simulink model "AirplaneSimModel_SITL_gazebo"  (R2018b)
settings: Solver=ode2  StartTime=0.0  StopTime=inf  FixedStep=0.0025  RelTol=1e-3
undefined symbols (not defined in the file): aileron_left, aileron_right, airplane, alt_ground, atmosphere, elevator, envir, g, htp_trim, rudder, throttle, wind
libraries: unit_conversions_lib x4, ardupilot_sitl_lib x2, conventional_airplane_single_engine_lib x1, atmosphere_lib x1, sensors_lib x1, simulink x1, flightgear_visualization_lib x1
settings Model: Creator=Yannic  LastModifiedBy=yannic
settings OptimizationCC: EfficientMapNaN2IntZero=off
settings HardwareCC: TargetBitPerLong=64  TargetBitPerPointer=64  TargetBitPerSizeT=64  TargetBitPerPtrDiffT=64  TargetLongLongMode=on  TargetIntDivRoundTo=Zero  TargetEndianess=LittleEndian  TargetWordSize=64  TargetHWDeviceType=MATLAB Host  ProdEqTarget=off
settings RTWCC: SystemTargetFile=rsim.tlc  TemplateMakefile=rsim_default_tmf  Description=Rapid Simulation Target  TargetLang=C++  RTWCompilerOptimization=on
settings CodeAppCC: MaxIdLength=128
settings RSimTargetCC: TargetLangStandard=C++03 (ISO)  GeneratePreprocessorConditionals=Use local settings  PreserveStateflowLocalDataDimensions=off

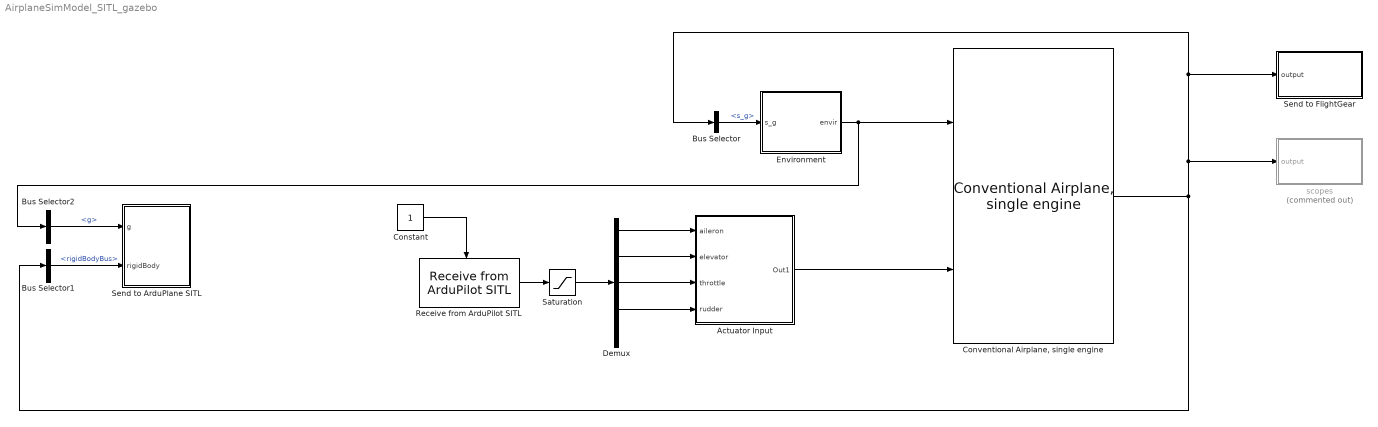
== system AirplaneSimModel_SITL_gazebo ==
  Actuator Input : Subsystem
  Bus Selector : BusSelector  OutputSignals=rigidBodyBus.s_g
  Bus Selector1 : BusSelector  OutputSignals=rigidBodyBus
  Bus Selector2 : BusSelector  OutputSignals=g
  Constant : Constant
  "Conventional Airplane, single engine" : conventional_airplane_single_engine_lib/Conventional Airplane, single engine  airplane=airplane
      settings: SourceProductName=LADAC
  Demux : Demux  Outputs=5
  Environment : Subsystem
  Receive from ArduPilot SITL : ardupilot_sitl_lib/Receive from ArduPilot SITL  idx=[1,2,3,4,5]  IP='127.0.0.1'  Port=9002  sample_time=1/400  blocking_time=1
      settings: SourceProductName=LADAC
  Saturation : Saturate  UpperLimit=1  LowerLimit=0
  Send to ArduPlane SITL : Subsystem
  Send to FlightGear : Subsystem
  scopes : Subsystem  Commented=on
  wires:
  Environment/1(envir) -> Bus Selector2/1, "Conventional Airplane, single engine"/1
  "Conventional Airplane, single engine"/1 -> Bus Selector1/1, Bus Selector/1, Send to FlightGear/1(output), scopes/1(output)
  Bus Selector/1 -> Environment/1(s_g)  "<s_g>"
  Bus Selector1/1 -> Send to ArduPlane SITL/2(rigidBody)  "<rigidBodyBus>"
  Bus Selector2/1 -> Send to ArduPlane SITL/1(g)  "<g>"
  Actuator Input/1(Out1) -> "Conventional Airplane, single engine"/2
  Demux/1 -> Actuator Input/1(aileron)
  Demux/4 -> Actuator Input/4(rudder)
  Receive from ArduPilot SITL/1 -> Saturation/1
  Constant/1 -> Receive from ArduPilot SITL/Enable
  Demux/2 -> Actuator Input/2(elevator)
  Demux/3 -> Actuator Input/3(throttle)
  Saturation/1 -> Demux/1

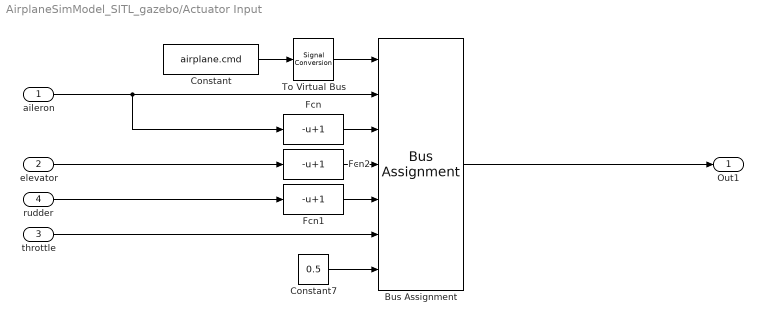
== system AirplaneSimModel_SITL_gazebo/Actuator Input ==
  aileron : Inport
  elevator : Inport  Port=2
  throttle : Inport  Port=3
  rudder : Inport  Port=4
  Bus Assignment : BusAssignment  AssignedSignals=aileron_left,aileron_right,elevator,rudder,throttle,htp_trim
  Constant : Constant  Value=airplane.cmd  OutDataTypeStr=Bus: cmdBus
  Constant7 : Constant  Value=0.5
  Fcn : Fcn  Expr=-u+1
  Fcn1 : Fcn  Expr=-u+1
  Fcn2 : Fcn  Expr=-u+1
  To Virtual Bus : SignalConversion  ConversionOutput=Virtual bus  OverrideOpt=off
  Out1 : Outport
  wires:
  Constant/1 -> To Virtual Bus/1
  Bus Assignment/1 -> Out1/1
  rudder/1 -> Fcn1/1
  elevator/1 -> Fcn2/1
  aileron/1 -> Fcn/1, Bus Assignment/2
  Constant7/1 -> Bus Assignment/7
  Fcn/1 -> Bus Assignment/3
  Fcn1/1 -> Bus Assignment/5
  To Virtual Bus/1 -> Bus Assignment/1
  throttle/1 -> Bus Assignment/6
  Fcn2/1 -> Bus Assignment/4

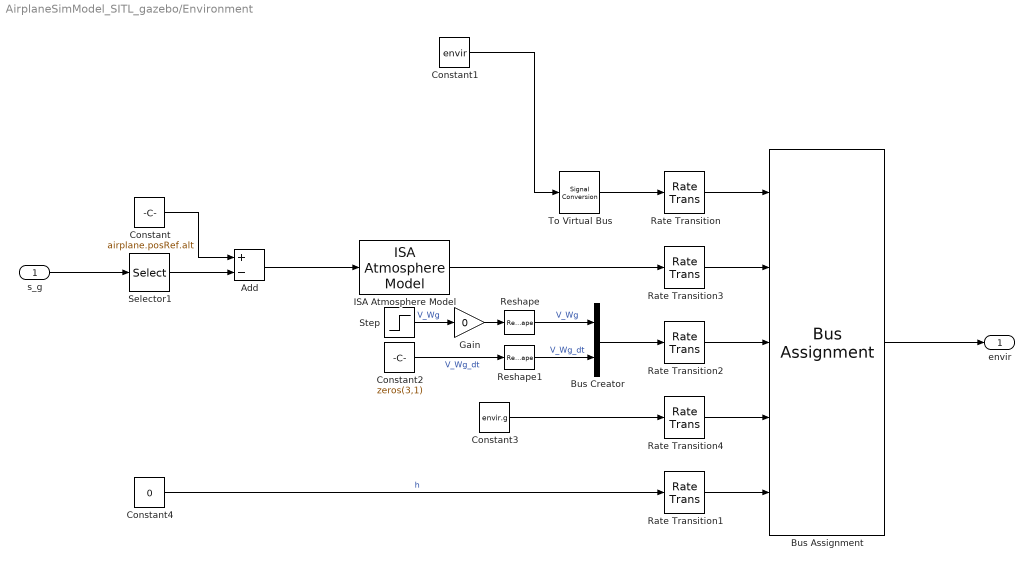
== system AirplaneSimModel_SITL_gazebo/Environment ==
  s_g : Inport
  Add : Sum  Inputs=+-
  Bus Assignment : BusAssignment  AssignedSignals=atmosphere,wind,g,alt_ground
  Bus Creator : BusCreator  Inputs=2
  Constant : Constant  Value=airplane.posRef.alt
  Constant1 : Constant  Value=envir  OutDataTypeStr=Bus: envirBus
  Constant2 : Constant  Value=zeros(3,1)
  Constant3 : Constant  Value=envir.g
  Constant4 : Constant  Value=0
  Gain : Gain  Gain=0
  ISA Atmosphere Model : atmosphere_lib/ISA Atmosphere Model
      settings: SourceProductName=LADAC
  Rate Transition{,1..4} (5 alike) : RateTransition
  Reshape : Reshape  OutputDimensionality=Column vector (2-D)
  Reshape1 : Reshape  OutputDimensionality=Column vector (2-D)
  Selector1 : Selector  InputPortWidth=3  IndexOptions=Index vector (dialog)  Indices=3  OutputSizes=1
  Step : Step  Time=3  After=[0;10;0]  SampleTime=0
  To Virtual Bus : SignalConversion  ConversionOutput=Virtual bus  OverrideOpt=off
  envir : Outport
  wires:
  Constant4/1 -> Rate Transition1/1  "h"
  Rate Transition2/1 -> Bus Assignment/3
  Rate Transition3/1 -> Bus Assignment/2
  Bus Assignment/1 -> envir/1
  Rate Transition/1 -> Bus Assignment/1
  ISA Atmosphere Model/1 -> Rate Transition3/1
  Step/1 -> Gain/1  "V_Wg"
  Rate Transition1/1 -> Bus Assignment/5
  s_g/1 -> Selector1/1
  Bus Creator/1 -> Rate Transition2/1
  Constant2/1 -> Reshape1/1  "V_Wg_dt"
  Rate Transition4/1 -> Bus Assignment/4
  Constant3/1 -> Rate Transition4/1
  Gain/1 -> Reshape/1
  Constant/1 -> Add/1
  Add/1 -> ISA Atmosphere Model/1
  Selector1/1 -> Add/2
  To Virtual Bus/1 -> Rate Transition/1
  Reshape/1 -> Bus Creator/1  "V_Wg"
  Reshape1/1 -> Bus Creator/2  "V_Wg_dt"
  Constant1/1 -> To Virtual Bus/1

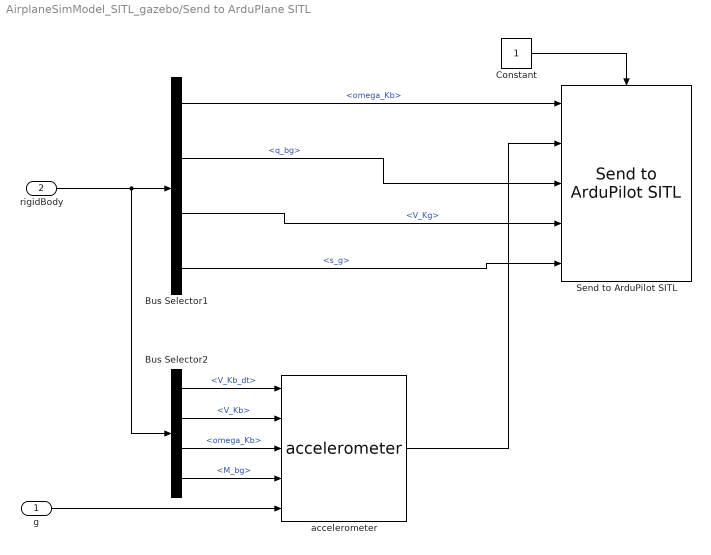
== system AirplaneSimModel_SITL_gazebo/Send to ArduPlane SITL ==
  g : Inport
  rigidBody : Inport  Port=2
  Bus Selector1 : BusSelector  OutputSignals=omega_Kb,q_bg,V_Kg,s_g
  Bus Selector2 : BusSelector  OutputSignals=V_Kb_dt,V_Kb,omega_Kb,M_bg
  Constant : Constant
  Send to ArduPilot SITL : ardupilot_sitl_lib/Send to ArduPilot SITL  IP='127.0.0.1'  Port=9003  sample_time=1/400
      settings: SourceProductName=LADAC
  accelerometer : sensors_lib/accelerometer  SystemSampleTime=-1
      settings: SourceProductName=LADAC
  wires:
  g/1 -> accelerometer/5
  Bus Selector1/4 -> Send to ArduPilot SITL/5  "<s_g>"
  Bus Selector1/2 -> Send to ArduPilot SITL/3  "<q_bg>"
  Bus Selector1/1 -> Send to ArduPilot SITL/1  "<omega_Kb>"
  rigidBody/1 -> Bus Selector2/1, Bus Selector1/1
  Bus Selector1/3 -> Send to ArduPilot SITL/4  "<V_Kg>"
  Constant/1 -> Send to ArduPilot SITL/Enable
  Bus Selector2/1 -> accelerometer/1  "<V_Kb_dt>"
  Bus Selector2/2 -> accelerometer/2  "<V_Kb>"
  Bus Selector2/3 -> accelerometer/3  "<omega_Kb>"
  Bus Selector2/4 -> accelerometer/4  "<M_bg>"
  accelerometer/1 -> Send to ArduPilot SITL/2

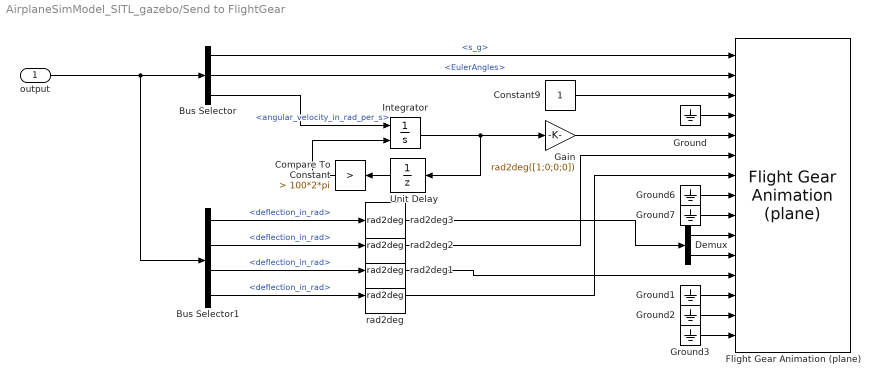
== system AirplaneSimModel_SITL_gazebo/Send to FlightGear ==
  output : Inport
  Bus Selector : BusSelector  OutputSignals=rigidBodyBus.s_g,rigidBodyBus.EulerAngles,actuatorBus.motorBus.angular_velocity_in_rad_per_s
  Bus Selector1 : BusSelector  OutputSignals=actuatorBus.aileronsBus.deflection_in_rad,actuatorBus.elevatorBus.deflection_in_rad,actuatorBus.rudderBus.deflection_in_rad,actuatorBus.htpTrimBus.deflection_in_rad
  Compare To Constant : simulink/Logic and Bit Operations/Compare To Constant  relop=>  const=100*2*pi  OutDataTypeStr=boolean
  Constant9 : Constant
  Demux : Demux  Outputs=2
  Flight Gear Animation (plane) : flightgear_visualization_lib/Flight Gear Animation (plane)  inital_lat=airplane.posRef.lat  inital_long=airplane.posRef.lon  inital_height=airplane.posRef.alt  remoteURL='127.0.0.1'  remotePort=5502
      settings: SourceProductName=LADAC
  Gain : Gain  Gain=rad2deg([1;0;0;0])
  Ground{,1..3,6..7} (6 alike) : Ground
  Integrator : Integrator  ExternalReset=rising
  Unit Delay : UnitDelay  SampleTime=-1
  rad2deg{,1..3} (4 alike) : unit_conversions_lib/rad2deg
      settings: SourceProductName=LADAC
  wires:
  Compare To Constant/1 -> Integrator/2
  Integrator/1 -> Unit Delay/1, Gain/1
  Bus Selector/1 -> Flight Gear Animation (plane)/1  "<s_g>"
  Bus Selector/2 -> Flight Gear Animation (plane)/2  "<EulerAngles>"
  Gain/1 -> Flight Gear Animation (plane)/5
  Constant9/1 -> Flight Gear Animation (plane)/3
  Unit Delay/1 -> Compare To Constant/1
  Ground/1 -> Flight Gear Animation (plane)/4
  Ground1/1 -> Flight Gear Animation (plane)/13
  Ground2/1 -> Flight Gear Animation (plane)/14
  Ground3/1 -> Flight Gear Animation (plane)/15
  output/1 -> Bus Selector1/1, Bus Selector/1
  Bus Selector/3 -> Integrator/1  "<angular_velocity_in_rad_per_s>"
  Bus Selector1/2 -> rad2deg2/1  "<deflection_in_rad>"
  Bus Selector1/4 -> rad2deg/1  "<deflection_in_rad>"
  Ground6/1 -> Flight Gear Animation (plane)/8
  Ground7/1 -> Flight Gear Animation (plane)/9
  Bus Selector1/3 -> rad2deg1/1  "<deflection_in_rad>"
  Bus Selector1/1 -> rad2deg3/1  "<deflection_in_rad>"
  Demux/1 -> Flight Gear Animation (plane)/10
  Demux/2 -> Flight Gear Animation (plane)/11
  rad2deg/1 -> Flight Gear Animation (plane)/7
  rad2deg1/1 -> Flight Gear Animation (plane)/12
  rad2deg2/1 -> Flight Gear Animation (plane)/6
  rad2deg3/1 -> Demux/1

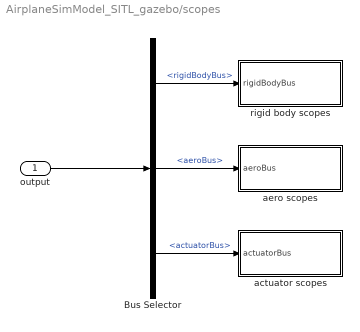
== system AirplaneSimModel_SITL_gazebo/scopes ==
  output : Inport
  Bus Selector : BusSelector  OutputSignals=rigidBodyBus,aeroBus,actuatorBus
  actuator scopes : Subsystem
  aero scopes : Subsystem
  rigid body scopes : Subsystem
  wires:
  Bus Selector/1 -> rigid body scopes/1(rigidBodyBus)  "<rigidBodyBus>"
  Bus Selector/2 -> aero scopes/1(aeroBus)  "<aeroBus>"
  output/1 -> Bus Selector/1
  Bus Selector/3 -> actuator scopes/1(actuatorBus)  "<actuatorBus>"

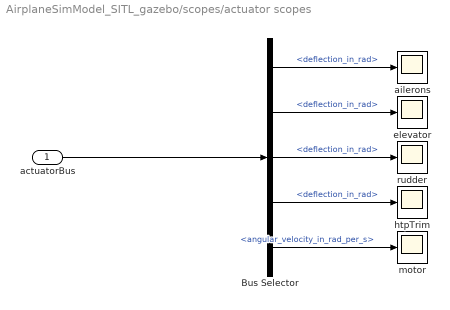
== system AirplaneSimModel_SITL_gazebo/scopes/actuator scopes ==
  actuatorBus : Inport
  Bus Selector : BusSelector  OutputSignals=aileronsBus.deflection_in_rad,elevatorBus.deflection_in_rad,rudderBus.deflection_in_rad,htpTrimBus.deflection_in_rad,motorBus.angular_velocity_in_rad_per_s
  ailerons : Scope
  elevator : Scope
  htpTrim : Scope
  motor : Scope
  rudder : Scope
  wires:
  actuatorBus/1 -> Bus Selector/1
  Bus Selector/1 -> ailerons/1  "<deflection_in_rad>"
  Bus Selector/2 -> elevator/1  "<deflection_in_rad>"
  Bus Selector/3 -> rudder/1  "<deflection_in_rad>"
  Bus Selector/4 -> htpTrim/1  "<deflection_in_rad>"
  Bus Selector/5 -> motor/1  "<angular_velocity_in_rad_per_s>"

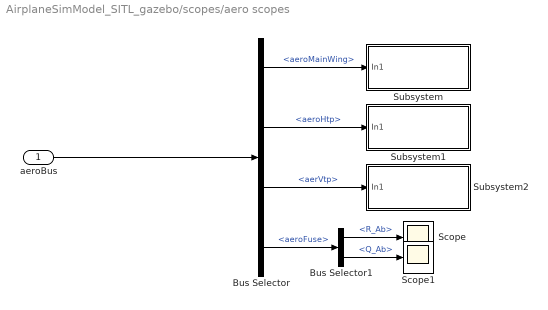
== system AirplaneSimModel_SITL_gazebo/scopes/aero scopes ==
  aeroBus : Inport
  Bus Selector : BusSelector  OutputSignals=aeroMainWing,aeroHtp,aerVtp,aeroFuse
  Bus Selector1 : BusSelector  OutputSignals=R_Ab,Q_Ab
  Scope : Scope
  Scope1 : Scope
  Subsystem : Subsystem
  Subsystem1 : Subsystem
  Subsystem2 : Subsystem
  wires:
  aeroBus/1 -> Bus Selector/1
  Bus Selector/1 -> Subsystem/1(In1)  "<aeroMainWing>"
  Bus Selector/2 -> Subsystem1/1(In1)  "<aeroHtp>"
  Bus Selector/3 -> Subsystem2/1(In1)  "<aerVtp>"
  Bus Selector/4 -> Bus Selector1/1  "<aeroFuse>"
  Bus Selector1/1 -> Scope/1  "<R_Ab>"
  Bus Selector1/2 -> Scope1/1  "<Q_Ab>"

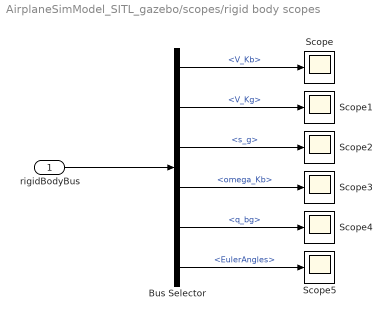
== system AirplaneSimModel_SITL_gazebo/scopes/rigid body scopes ==
  rigidBodyBus : Inport
  Bus Selector : BusSelector  OutputSignals=V_Kb,V_Kg,s_g,omega_Kb,q_bg,EulerAngles
  Scope{,1..5} (6 alike) : Scope
  wires:
  rigidBodyBus/1 -> Bus Selector/1
  Bus Selector/1 -> Scope/1  "<V_Kb>"
  Bus Selector/2 -> Scope1/1  "<V_Kg>"
  Bus Selector/3 -> Scope2/1  "<s_g>"
  Bus Selector/4 -> Scope3/1  "<omega_Kb>"
  Bus Selector/5 -> Scope4/1  "<q_bg>"
  Bus Selector/6 -> Scope5/1  "<EulerAngles>"

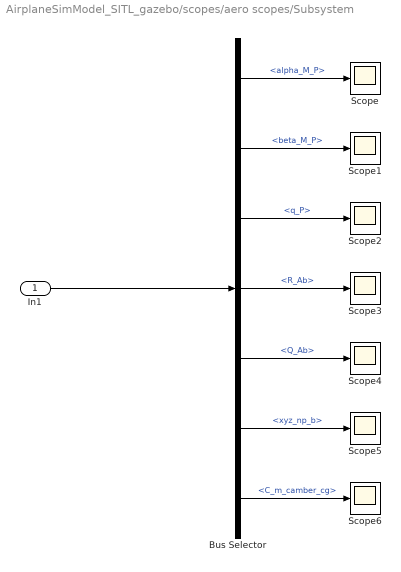
== system AirplaneSimModel_SITL_gazebo/scopes/aero scopes/Subsystem ==
  In1 : Inport
  Bus Selector : BusSelector  OutputSignals=aeroAxes.alpha_M_P,aeroAxes.beta_M_P,aeroAxes.q_P,dynamics.R_Ab,dynamics.Q_Ab,dynamics.xyz_np_b,dynamics.C_m_camber_cg
  Scope{,1..6} (7 alike) : Scope
  wires:
  In1/1 -> Bus Selector/1
  Bus Selector/1 -> Scope/1  "<alpha_M_P>"
  Bus Selector/3 -> Scope2/1  "<q_P>"
  Bus Selector/2 -> Scope1/1  "<beta_M_P>"
  Bus Selector/4 -> Scope3/1  "<R_Ab>"
  Bus Selector/5 -> Scope4/1  "<Q_Ab>"
  Bus Selector/6 -> Scope5/1  "<xyz_np_b>"
  Bus Selector/7 -> Scope6/1  "<C_m_camber_cg>"

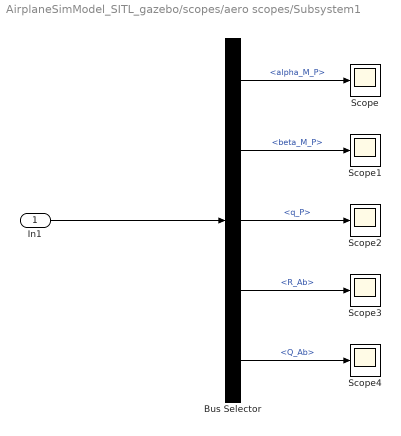
== system AirplaneSimModel_SITL_gazebo/scopes/aero scopes/Subsystem1 ==
  In1 : Inport
  Bus Selector : BusSelector  OutputSignals=aeroAxes.alpha_M_P,aeroAxes.beta_M_P,aeroAxes.q_P,dynamics.R_Ab,dynamics.Q_Ab
  Scope{,1..4} (5 alike) : Scope
  wires:
  Bus Selector/5 -> Scope4/1  "<Q_Ab>"
  Bus Selector/4 -> Scope3/1  "<R_Ab>"
  Bus Selector/2 -> Scope1/1  "<beta_M_P>"
  Bus Selector/3 -> Scope2/1  "<q_P>"
  Bus Selector/1 -> Scope/1  "<alpha_M_P>"
  In1/1 -> Bus Selector/1

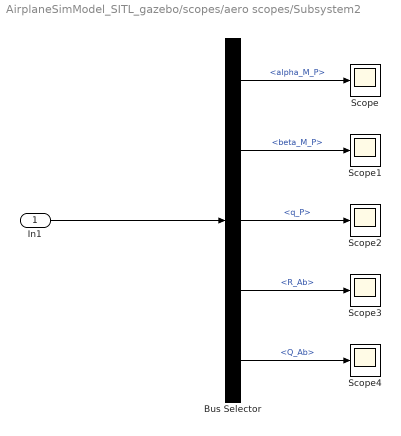
== system AirplaneSimModel_SITL_gazebo/scopes/aero scopes/Subsystem2 ==
  In1 : Inport
  Bus Selector : BusSelector  OutputSignals=aeroAxes.alpha_M_P,aeroAxes.beta_M_P,aeroAxes.q_P,dynamics.R_Ab,dynamics.Q_Ab
  Scope{,1..4} (5 alike) : Scope
  wires:
  In1/1 -> Bus Selector/1
  Bus Selector/1 -> Scope/1  "<alpha_M_P>"
  Bus Selector/3 -> Scope2/1  "<q_P>"
  Bus Selector/2 -> Scope1/1  "<beta_M_P>"
  Bus Selector/4 -> Scope3/1  "<R_Ab>"
  Bus Selector/5 -> Scope4/1  "<Q_Ab>"
